simulink model "MicrogridAverage"  (R2026a)
settings: Solver=ode23t  StopTime=5  MaxStep=0.0001  RelTol=1e-4
model workspace (MAT data in the model file):
  mgIrradiance = [0  800; 1.5  800; 1.7  200; 5  200]
  mgLoadPower = [0  20000; 3.5  20000; 3.51  35000; 5  35000]
libraries: nesl_utility x20, fl_lib x9, ee_lib x8, greenH2_lib x5, batteryecm_lib x1
settings Model: Creator=LENOVO  LastModifiedBy=LENOVO
settings SimscapeCC: SimscapeLogDecimation=10.0  SimscapeLogLimitData=off

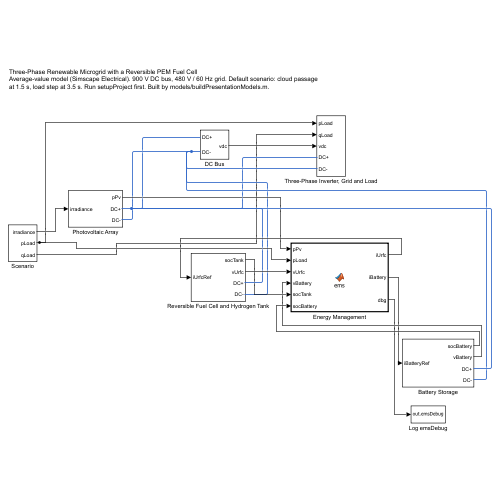
[thumbnail: Simulink's stored preview of the top-level diagram]
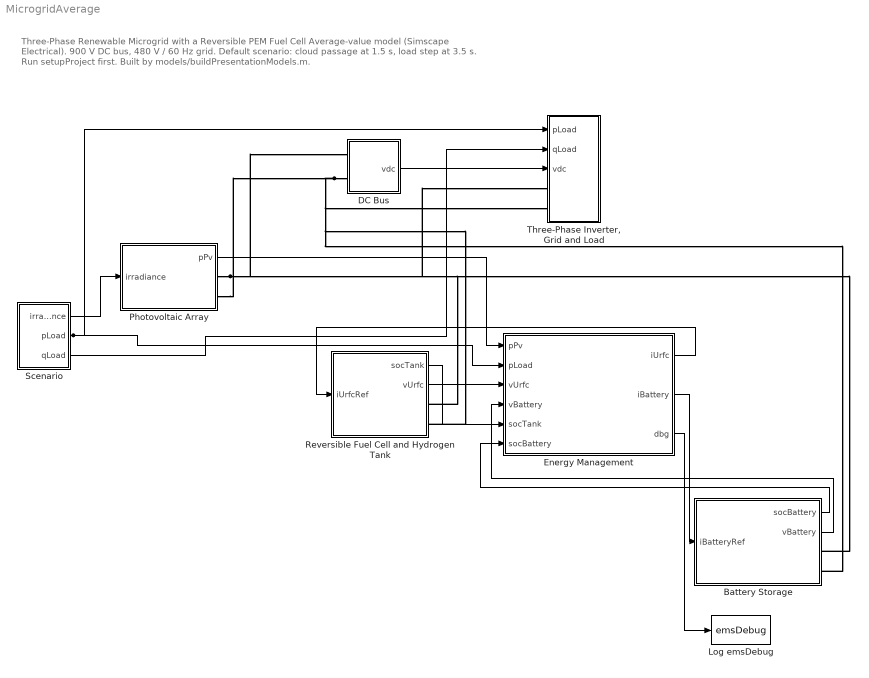
== system MicrogridAverage ==
  note: Three-Phase Renewable Microgrid with a Reversible PEM Fuel Cell
      | Average-value model (Simscape Electrical). 900 V DC bus, 480 V / 60 Hz grid. Default scenario: cloud passage
      | at 1.5 s, load step at 3.5 s. Run setupProject first. Built by models/buildPresentationModels.m.
  Battery Storage : Subsystem
  DC Bus : Subsystem
  Energy Management : MATLAB Function  TreatAsAtomicUnit=on
  Log emsDebug : ToWorkspace  VariableName=emsDebug  SaveFormat=Timeseries  SampleTime=-1
  Photovoltaic Array : Subsystem
  Reversible Fuel Cell and Hydrogen Tank : Subsystem
  Scenario : Subsystem
  "Three-Phase Inverter, Grid and Load" : Subsystem
  wires:
  Scenario/1(irradiance) -> Photovoltaic Array/1(irradiance)
  Scenario/2(pLoad) -> Energy Management/2(pLoad), "Three-Phase Inverter, Grid and Load"/1(pLoad)
  Scenario/3(qLoad) -> "Three-Phase Inverter, Grid and Load"/2(qLoad)
  DC Bus/1(vdc) -> "Three-Phase Inverter, Grid and Load"/3(vdc)
  Photovoltaic Array/1(pPv) -> Energy Management/1(pPv)
  Reversible Fuel Cell and Hydrogen Tank/1(socTank) -> Energy Management/5(socTank)
  Reversible Fuel Cell and Hydrogen Tank/2(vUrfc) -> Energy Management/3(vUrfc)
  Energy Management/1(iUrfc) -> Reversible Fuel Cell and Hydrogen Tank/1(iUrfcRef)
  Battery Storage/2(vBattery) -> Energy Management/4(vBattery)
  Energy Management/2(iBattery) -> Battery Storage/1(iBatteryRef)
  Energy Management/3(dbg) -> Log emsDebug/1
  Battery Storage/1(socBattery) -> Energy Management/6(socBattery)
  connections:
  Photovoltaic Array/RConn2 -- Reversible Fuel Cell and Hydrogen Tank/RConn2 -- "Three-Phase Inverter, Grid and Load"/LConn2 -- Battery Storage/RConn2 -- DC Bus/LConn2
  Photovoltaic Array/RConn1 -- Reversible Fuel Cell and Hydrogen Tank/RConn1 -- Battery Storage/RConn1 -- "Three-Phase Inverter, Grid and Load"/LConn1 -- DC Bus/LConn1

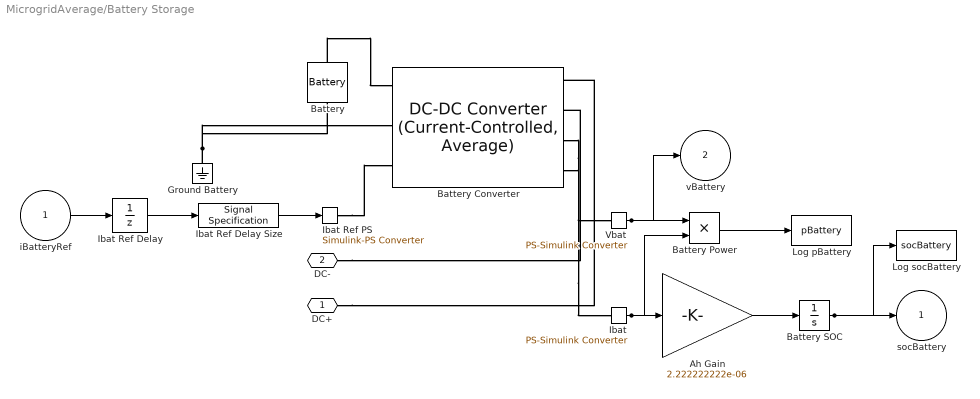
== system MicrogridAverage/Battery Storage ==
  iBatteryRef : Inport
  Ah Gain : Gain  Gain=2.222222222e-06
  Battery : batteryecm_lib/Battery  Vnom=400 V  prm_dir=simscape.enum.battery.prm_dir.disabled  R1_dis=2 Ohm  R1_ch=2 Ohm  R1=0.08 Ohm  prm_AH=simscape.enum.battery.prm_AH.finite  AH=125 A*hr  V1=380 V  AH1=62.5 A*hr  prm_R2=simscape.enum.battery.prm_R2.disabled  R2=2000 Ohm  Tmeas=298.15 K  charge_measurement_port=simscape.enum.battery.enable.no  prm_dyn=simscape.enum.battery.prm_dyn.off  Rp1=0.005 Ohm  tau1=30 s  Rp2=0.005 Ohm  tau2=30 s  Rp3=0.005 Ohm  tau3=30 s  Rp4=0.005 Ohm  tau4=30 s  Rp5=0.005 Ohm  tau5=30 s  prm_fade=simscape.enum.battery.prm_fade.disabled  N_fade=100  AH_fade=45 A*hr  R1_fade=2.02 Ohm  R1_ch_fade=2.02 Ohm  V1_fade=10.35 V  prm_age=simscape.enum.battery.prm_age.disabled  prm_age_OCV=simscape.enum.battery.prm_age_OCV.OCV  OCV_age=0.9  SOC_age=60  Tmeas_age=298.15 K  delta_time_age_vec=[0] d  temperature_age_vec=[273] K  OCV_scaling_age=2.2134e6  OCV_offset_age=1.632e6  temp_exp_age=0.515833569 V  t_exp_age=0.75  Vnom_T2=12 V  R1_T2=2.2 Ohm  R1_T2_dis=2.2 Ohm  R1_T2_ch=2.2 Ohm  V1_T2=11.4 V  R2_T2=2200 Ohm  Rp1_T2=0.005 Ohm  tau1_T2=30 s  Rp2_T2=0.005 Ohm  tau2_T2=30 s  Rp3_T2=0.005 Ohm  tau3_T2=30 s  Rp4_T2=0.005 Ohm  tau4_T2=30 s  Rp5_T2=0.005 Ohm  tau5_T2=30 s  Tmeas2=273.15 K  thermal_port=simscape.enum.thermaleffects.omit  thermal_mass=30000 J/K  i_specify=off  i_priority=None  i=0 A  i_nominal_specify=off  i_nominal_value=1  i_nominal_unit=A  v_specify=off  v_priority=None  v=0 V  v_nominal_specify=off  v_nominal_value=1  v_nominal_unit=V  charge_specify=off  charge_priority=High  charge=50 A*hr  charge_nominal_specify=off  charge_nominal_value=1  charge_nominal_unit=A*hr  num_cycles_specify=off  num_cycles_priority=High  num_cycles=0  num_cycles_nominal_specify=off  num_cycles_nominal_value=1  num_cycles_nominal_unit=1  temperature_specify=off  temperature_priority=High  temperature=298.15 K  temperature_nominal_specify=off  temperature_nominal_value=1  temperature_nominal_unit=K
  Battery Converter : greenH2_lib/DC-DC Converter (Current-Controlled, Average)  eta=0.97  v_min=10 V  i1_specify=off  i1_priority=None  i1=0 A  i1_nominal_specify=off  i1_nominal_value=1  i1_nominal_unit=A  i2_specify=off  i2_priority=None  i2=0 A  i2_nominal_specify=off  i2_nominal_value=1  i2_nominal_unit=A
  Battery Power : Product
  Battery SOC : Integrator  InitialCondition=0.6
  Ground Battery : fl_lib/Electrical/Electrical Elements/Electrical Reference
  Ibat : nesl_utility/PS-Simulink Converter  PhysicalDomain=network_engine_domain  SubClassName=ps_output  LeftPortType=input  RightPortType=output  PseudoPeriodic=off  Frequencies=[]  VectorFormat=inherit  Unit=A  AffineConversion=off
  Ibat Ref Delay : UnitDelay  SampleTime=0.001
  Ibat Ref Delay Size : SignalSpecification  Dimensions=1
  Ibat Ref PS : nesl_utility/Simulink-PS Converter  PhysicalDomain=network_engine_domain  SubClassName=ps_input  LeftPortType=input  RightPortType=output  PseudoPeriodic=off  Frequencies=[]  NoiseDistribution=none  NoiseParameters=[]  Unit=A  AffineConversion=off  FilteringAndDerivatives=provide  SimscapeFilterOrder=1  InputFilterTimeConstant=0.001  UdotUserProvided=0
  Log pBattery : ToWorkspace  VariableName=pBattery  SaveFormat=Timeseries  SampleTime=-1
  Log socBattery : ToWorkspace  VariableName=socBattery  SaveFormat=Timeseries  SampleTime=-1
  Vbat : nesl_utility/PS-Simulink Converter  PhysicalDomain=network_engine_domain  SubClassName=ps_output  LeftPortType=input  RightPortType=output  PseudoPeriodic=off  Frequencies=[]  VectorFormat=inherit  Unit=V  AffineConversion=off
  DC+ : PMIOPort  Side=Right
  DC- : PMIOPort  Port=2  Side=Right
  socBattery : Outport
  vBattery : Outport  Port=2
  wires:
  iBatteryRef/1 -> Ibat Ref Delay/1
  Ibat Ref Delay/1 -> Ibat Ref Delay Size/1
  Vbat/1 -> Battery Power/1, vBattery/1
  Ibat Ref Delay Size/1 -> Ibat Ref PS/1
  Ah Gain/1 -> Battery SOC/1
  Ibat/1 -> Ah Gain/1, Battery Power/2
  Battery Power/1 -> Log pBattery/1
  Battery SOC/1 -> socBattery/1, Log socBattery/1
  connections:
  Ground Battery/LConn1 -- Battery/RConn1 -- Battery Converter/LConn2
  Ibat Ref PS/RConn1 -- Battery Converter/LConn3
  Battery/LConn1 -- Battery Converter/LConn1
  DC-/RConn1 -- Battery Converter/RConn2
  DC+/RConn1 -- Battery Converter/RConn1
  Battery Converter/RConn4 -- Ibat/LConn1
  Battery Converter/RConn3 -- Vbat/LConn1

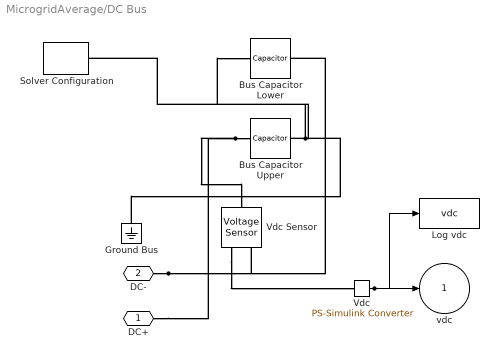
== system MicrogridAverage/DC Bus ==
  Bus Capacitor Lower : fl_lib/Electrical/Electrical Elements/Capacitor  c=0.01 F  r=1e-6 Ohm  g=0 1/Ohm  i_specify=off  i_priority=None  i=0 A  i_nominal_specify=off  i_nominal_value=1  i_nominal_unit=A  v_specify=off  v_priority=None  v=0 V  v_nominal_specify=off  v_nominal_value=1  v_nominal_unit=V  vc_specify=on  vc_priority=High  vc=450 V  vc_nominal_specify=off  vc_nominal_value=1  vc_nominal_unit=V
  Bus Capacitor Upper : fl_lib/Electrical/Electrical Elements/Capacitor  c=0.01 F  r=1e-6 Ohm  g=0 1/Ohm  i_specify=off  i_priority=None  i=0 A  i_nominal_specify=off  i_nominal_value=1  i_nominal_unit=A  v_specify=off  v_priority=None  v=0 V  v_nominal_specify=off  v_nominal_value=1  v_nominal_unit=V  vc_specify=on  vc_priority=High  vc=450 V  vc_nominal_specify=off  vc_nominal_value=1  vc_nominal_unit=V
  Ground Bus : fl_lib/Electrical/Electrical Elements/Electrical Reference
  Log vdc : ToWorkspace  VariableName=vdc  SaveFormat=Timeseries  SampleTime=-1
  Solver Configuration : nesl_utility/Solver Configuration  PhysicalDomain=network_engine_domain  SubClassName=solver  LeftPortType=input  RightPortType=generic  Tones=[]  Harmonics=[]  SimulateNoise=off  Profile=off  UseLocalSampling=off  EnableSwitchedLinearOptims=on  FrequencyDomain=off  UseCCode=off  RelTol=0.001  AbsTol=0.001  MinStep=1e-09  ToWorkspace=off  RevertToSquareIcSolve=off  NumHomotopyIterations=100  PhasorMode=off  PhasorModeNumHarmonics=1  ConsistencySolver=NEWTON_XTOL_AFTER_FTOL  CanonicalOrdering=CANONICAL  OptimizeIntermediates=OPTIMIZED  IndexReductionMethod=DerivativeReplacement  DoDC=off  ResidualTolerance=1e-09  ConsistencyTolSource=GLOBAL  ConsistencyAbsTol=0.001  ConsistencyRelTol=0.001  ConsistencyTolFactor=0.001  UseLocalSolver=off  LocalSolverChoice=NE_BACKWARD_EULER_ADVANCER  ResolveIndetEquations=on  FunctionEvalNumThread=1  LocalSolverSampleTime=0.001  DoFixedCost=off  MaxNonlinIter=3  MaxModeIter=2  ComputeImpulses=off  ImpulseIterations=2  LinearAlgebra=auto  LinearAlgebraNumThread=0  EquationFormulation=NE_TIME_EF  DelaysMemoryBudget=1024  AutomaticFiltering=on  FilteringTimeConstant=0.001  PartitionStorageMethod=AS_NEEDED  PartitionMemoryBudget=1024  PartitionMethod=ROBUST  MultibodyUseLocalSolver=off  MultibodyLocalSolverChoice=ODE1  MultibodyLocalSolverSampleTime=0.001
  Vdc : nesl_utility/PS-Simulink Converter  PhysicalDomain=network_engine_domain  SubClassName=ps_output  LeftPortType=input  RightPortType=output  PseudoPeriodic=off  Frequencies=[]  VectorFormat=inherit  Unit=V  AffineConversion=off
  Vdc Sensor : fl_lib/Electrical/Electrical Sensors/Voltage Sensor
  DC+ : PMIOPort  Side=Left
  DC- : PMIOPort  Port=2  Side=Left
  vdc : Outport
  wires:
  Vdc/1 -> Log vdc/1, vdc/1
  connections:
  Ground Bus/LConn1 -- Solver Configuration/RConn1 -- Bus Capacitor Lower/LConn1 -- Bus Capacitor Upper/RConn1
  DC-/RConn1 -- Vdc Sensor/RConn2 -- Bus Capacitor Lower/RConn1
  DC+/RConn1 -- Vdc Sensor/LConn1 -- Bus Capacitor Upper/LConn1
  Vdc Sensor/RConn1 -- Vdc/LConn1

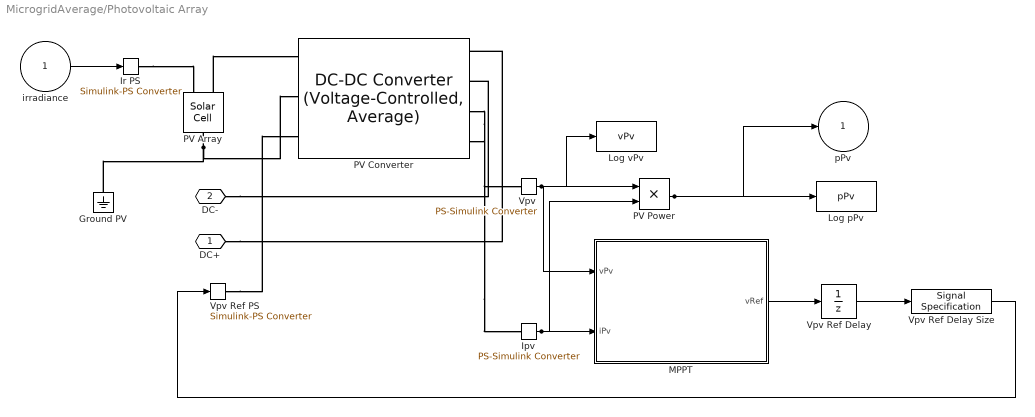
== system MicrogridAverage/Photovoltaic Array ==
  irradiance : Inport
  Ground PV : fl_lib/Electrical/Electrical Elements/Electrical Reference
  Ipv : nesl_utility/PS-Simulink Converter  PhysicalDomain=network_engine_domain  SubClassName=ps_output  LeftPortType=input  RightPortType=output  PseudoPeriodic=off  Frequencies=[]  VectorFormat=inherit  Unit=A  AffineConversion=off
  Ir PS : nesl_utility/Simulink-PS Converter  PhysicalDomain=network_engine_domain  SubClassName=ps_input  LeftPortType=input  RightPortType=output  PseudoPeriodic=off  Frequencies=[]  NoiseDistribution=none  NoiseParameters=[]  Unit=W/m^2  AffineConversion=off  FilteringAndDerivatives=provide  SimscapeFilterOrder=1  InputFilterTimeConstant=0.001  UdotUserProvided=0
  Log pPv : ToWorkspace  VariableName=pPv  SaveFormat=Timeseries  SampleTime=-1
  Log vPv : ToWorkspace  VariableName=vPv  SaveFormat=Timeseries  SampleTime=-1
  MPPT : MATLAB Function  TreatAsAtomicUnit=on
  PV Array : ee_lib/Sources/Solar Cell  prm=ee.enum.sources.solar_cell_prm.datasheet  Isc=9 A  Voc=0.6 V  Is=1e-6 A  Is2=0 A  Iph=7.34 A  Ir0=1000 W/m^2  ec=1.5  N2=2  Rs=0 Ohm  Rp=inf Ohm  N_series=1200  N_parallel=12  TIPH1=0 1/K  EG=1.11 eV  TXIS1=3  TXIS2=3  TRS1=0  TRP1=0  Tmeas=25 degC  TFIXED=25 degC  thermal_mass=100 J/K  initial_temperature=25 degC
  PV Converter : greenH2_lib/DC-DC Converter (Voltage-Controlled, Average)  eta=0.98  v_min=10 V  i1_specify=off  i1_priority=None  i1=0 A  i1_nominal_specify=off  i1_nominal_value=1  i1_nominal_unit=A  i2_specify=off  i2_priority=None  i2=0 A  i2_nominal_specify=off  i2_nominal_value=1  i2_nominal_unit=A
  PV Power : Product
  Vpv : nesl_utility/PS-Simulink Converter  PhysicalDomain=network_engine_domain  SubClassName=ps_output  LeftPortType=input  RightPortType=output  PseudoPeriodic=off  Frequencies=[]  VectorFormat=inherit  Unit=V  AffineConversion=off
  Vpv Ref Delay : UnitDelay  InitialCondition=570  SampleTime=0.01
  Vpv Ref Delay Size : SignalSpecification  Dimensions=1
  Vpv Ref PS : nesl_utility/Simulink-PS Converter  PhysicalDomain=network_engine_domain  SubClassName=ps_input  LeftPortType=input  RightPortType=output  PseudoPeriodic=off  Frequencies=[]  NoiseDistribution=none  NoiseParameters=[]  Unit=V  AffineConversion=off  FilteringAndDerivatives=provide  SimscapeFilterOrder=1  InputFilterTimeConstant=0.001  UdotUserProvided=0
  DC+ : PMIOPort  Side=Right
  DC- : PMIOPort  Port=2  Side=Right
  pPv : Outport
  wires:
  PV Power/1 -> pPv/1, Log pPv/1
  irradiance/1 -> Ir PS/1
  Vpv/1 -> MPPT/1(vPv), PV Power/1, Log vPv/1
  Ipv/1 -> MPPT/2(iPv), PV Power/2
  MPPT/1(vRef) -> Vpv Ref Delay/1
  Vpv Ref Delay/1 -> Vpv Ref Delay Size/1
  Vpv Ref Delay Size/1 -> Vpv Ref PS/1
  connections:
  Ground PV/LConn1 -- PV Array/RConn1 -- PV Converter/LConn2
  Ir PS/RConn1 -- PV Array/LConn1
  PV Array/LConn2 -- PV Converter/LConn1
  DC-/RConn1 -- PV Converter/RConn2
  DC+/RConn1 -- PV Converter/RConn1
  PV Converter/RConn4 -- Ipv/LConn1
  Vpv Ref PS/RConn1 -- PV Converter/LConn3
  PV Converter/RConn3 -- Vpv/LConn1

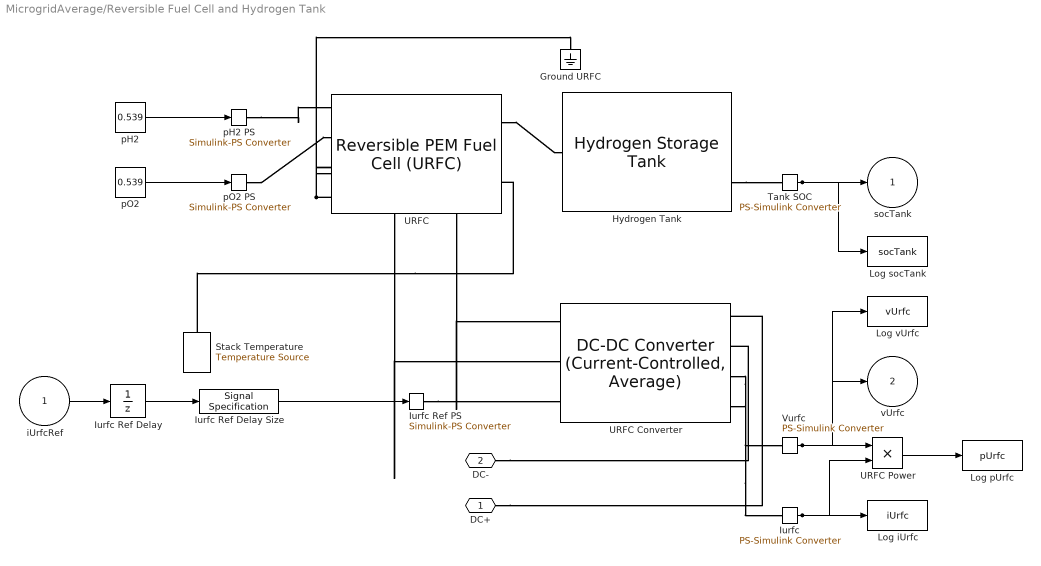
== system MicrogridAverage/Reversible Fuel Cell and Hydrogen Tank ==
  iUrfcRef : Inport
  Ground URFC : fl_lib/Electrical/Electrical Elements/Electrical Reference
  Hydrogen Tank : greenH2_lib/Hydrogen Storage Tank  V_tank=0.5 m^3  T_tank=298.15 K  p_init=30 bar  p_min=5 bar  p_max=350 bar  b_H2=1.55e-05 m^3/mol  n_specify=off  n_priority=None  n=1000 mol  n_nominal_specify=off  n_nominal_value=1  n_nominal_unit=mol
  Iurfc : nesl_utility/PS-Simulink Converter  PhysicalDomain=network_engine_domain  SubClassName=ps_output  LeftPortType=input  RightPortType=output  PseudoPeriodic=off  Frequencies=[]  VectorFormat=inherit  Unit=A  AffineConversion=off
  Iurfc Ref Delay : UnitDelay  SampleTime=0.001
  Iurfc Ref Delay Size : SignalSpecification  Dimensions=1
  Iurfc Ref PS : nesl_utility/Simulink-PS Converter  PhysicalDomain=network_engine_domain  SubClassName=ps_input  LeftPortType=input  RightPortType=output  PseudoPeriodic=off  Frequencies=[]  NoiseDistribution=none  NoiseParameters=[]  Unit=A  AffineConversion=off  FilteringAndDerivatives=provide  SimscapeFilterOrder=1  InputFilterTimeConstant=0.001  UdotUserProvided=0
  Log iUrfc : ToWorkspace  VariableName=iUrfc  SaveFormat=Timeseries  SampleTime=-1
  Log pUrfc : ToWorkspace  VariableName=pUrfc  SaveFormat=Timeseries  SampleTime=-1
  Log socTank : ToWorkspace  VariableName=socTank  SaveFormat=Timeseries  SampleTime=-1
  Log vUrfc : ToWorkspace  VariableName=vUrfc  SaveFormat=Timeseries  SampleTime=-1
  Stack Temperature : fl_lib/Thermal/Thermal Sources/Temperature Source  temperature=353.15 K
  Tank SOC : nesl_utility/PS-Simulink Converter  PhysicalDomain=network_engine_domain  SubClassName=ps_output  LeftPortType=input  RightPortType=output  PseudoPeriodic=off  Frequencies=[]  VectorFormat=inherit  Unit=1  AffineConversion=off
  URFC : greenH2_lib/Reversible PEM Fuel Cell (URFC)  N_cell=100  A_cell=300 cm^2  t_mem=0.0050800000000000003 cm  lambda_EC=22  lambda_FC=10.109999999999999  R_contact=0.037440000000000001 Ohm*cm^2  j0_EC=0.0001009 A/cm^2  alpha_EC=0.5  j0_FC=1.4800000000000001e-05 A/cm^2  alpha_FC=0.5  gamma_O2=0.75149999999999995  E_a=0 J/mol  T_ref=353.14999999999998 K  jL_EC=20 A/cm^2  jL_FC=17.780000000000001 A/cm^2  psi_H2=8.2000000000000001e-11 mol/(cm*s*bar)  i_specify=off  i_priority=None  i=0 A  i_nominal_specify=off  i_nominal_value=1  i_nominal_unit=A  Q_specify=off  Q_priority=None  Q=0 W  Q_nominal_specify=off  Q_nominal_value=1  Q_nominal_unit=W
  URFC Converter : greenH2_lib/DC-DC Converter (Current-Controlled, Average)  eta=0.97  v_min=10 V  i1_specify=off  i1_priority=None  i1=0 A  i1_nominal_specify=off  i1_nominal_value=1  i1_nominal_unit=A  i2_specify=off  i2_priority=None  i2=0 A  i2_nominal_specify=off  i2_nominal_value=1  i2_nominal_unit=A
  URFC Power : Product
  Vurfc : nesl_utility/PS-Simulink Converter  PhysicalDomain=network_engine_domain  SubClassName=ps_output  LeftPortType=input  RightPortType=output  PseudoPeriodic=off  Frequencies=[]  VectorFormat=inherit  Unit=V  AffineConversion=off
  pH2 : Constant  Value=0.539
  pH2 PS : nesl_utility/Simulink-PS Converter  PhysicalDomain=network_engine_domain  SubClassName=ps_input  LeftPortType=input  RightPortType=output  PseudoPeriodic=off  Frequencies=[]  NoiseDistribution=none  NoiseParameters=[]  Unit=bar  AffineConversion=off  FilteringAndDerivatives=provide  SimscapeFilterOrder=1  InputFilterTimeConstant=0.001  UdotUserProvided=0
  pO2 : Constant  Value=0.539
  pO2 PS : nesl_utility/Simulink-PS Converter  PhysicalDomain=network_engine_domain  SubClassName=ps_input  LeftPortType=input  RightPortType=output  PseudoPeriodic=off  Frequencies=[]  NoiseDistribution=none  NoiseParameters=[]  Unit=bar  AffineConversion=off  FilteringAndDerivatives=provide  SimscapeFilterOrder=1  InputFilterTimeConstant=0.001  UdotUserProvided=0
  DC+ : PMIOPort  Side=Right
  DC- : PMIOPort  Port=2  Side=Right
  socTank : Outport
  vUrfc : Outport  Port=2
  wires:
  Iurfc Ref Delay/1 -> Iurfc Ref Delay Size/1
  iUrfcRef/1 -> Iurfc Ref Delay/1
  pH2/1 -> pH2 PS/1
  pO2/1 -> pO2 PS/1
  Iurfc Ref Delay Size/1 -> Iurfc Ref PS/1
  Iurfc/1 -> Log iUrfc/1, URFC Power/2
  Tank SOC/1 -> socTank/1, Log socTank/1
  Vurfc/1 -> vUrfc/1, URFC Power/1, Log vUrfc/1
  URFC Power/1 -> Log pUrfc/1
  connections:
  URFC Converter/RConn3 -- Vurfc/LConn1
  URFC/LConn4 -- URFC Converter/LConn2 -- Ground URFC/LConn1
  pH2 PS/RConn1 -- URFC/LConn1
  DC-/RConn1 -- URFC Converter/RConn2
  pO2 PS/RConn1 -- URFC/LConn2
  URFC Converter/RConn4 -- Iurfc/LConn1
  Stack Temperature/LConn1 -- URFC/RConn2
  URFC/RConn1 -- Hydrogen Tank/LConn1
  URFC/LConn3 -- URFC Converter/LConn1
  Iurfc Ref PS/RConn1 -- URFC Converter/LConn3
  DC+/RConn1 -- URFC Converter/RConn1
  Hydrogen Tank/RConn2 -- Tank SOC/LConn1

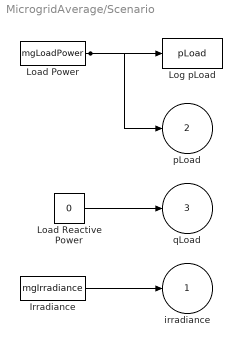
== system MicrogridAverage/Scenario ==
  Irradiance : FromWorkspace  VariableName=mgIrradiance  OutputAfterFinalValue=Holding final value
  Load Power : FromWorkspace  VariableName=mgLoadPower  OutputAfterFinalValue=Holding final value
  Load Reactive Power : Constant  Value=0
  Log pLoad : ToWorkspace  VariableName=pLoad  SaveFormat=Timeseries  SampleTime=-1
  irradiance : Outport
  pLoad : Outport  Port=2
  qLoad : Outport  Port=3
  wires:
  Irradiance/1 -> irradiance/1
  Load Power/1 -> pLoad/1, Log pLoad/1
  Load Reactive Power/1 -> qLoad/1

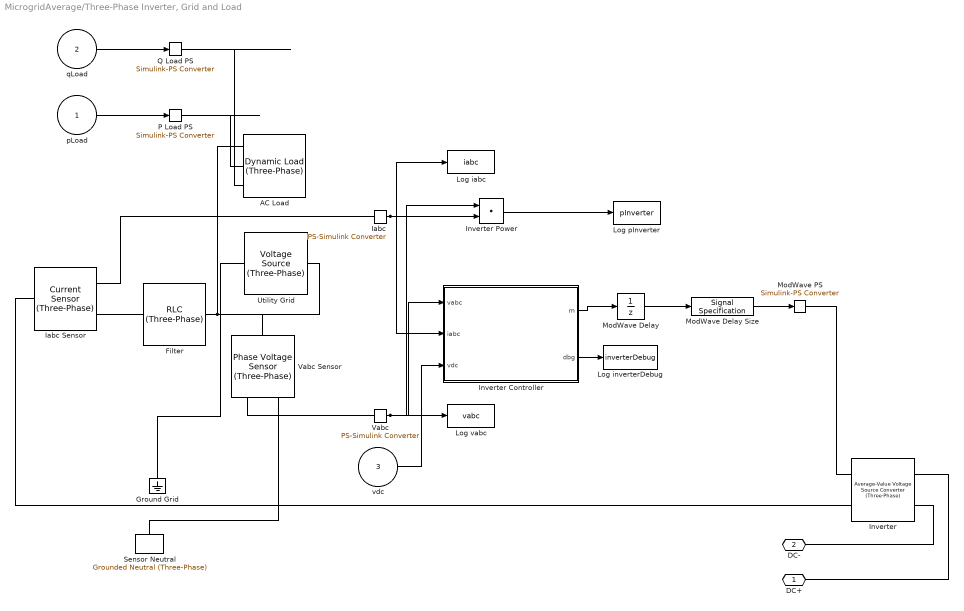
== system MicrogridAverage/Three-Phase Inverter, Grid and Load ==
  pLoad : Inport
  qLoad : Inport  Port=2
  vdc : Inport  Port=3
  AC Load : ee_lib/Passive/Dynamic Load (Three-Phase)  port_option=ee.enum.threePhasePort.composite  FRated=60 Hz  Vline_rms_min=240 V  tau=0.01 s  Vline_rms_ini=480 V  Vang_ini=0 deg  gmin=0 S
  Filter : ee_lib/Passive/RLC Assemblies/RLC (Three-Phase)  port_option=ee.enum.threePhasePort.composite  component_structure=ee.enum.rlc.structure.SeriesRL  R=0.05 Ohm  L=0.002 H  C=1e-6 F  R_parasitic=0 Ohm  G_parasitic=0 1/Ohm  IL_specify=off  IL_priority=High  IL=[0, 0, 0] A  IL_nominal_specify=off  IL_nominal_value=1  IL_nominal_unit=A  VC_specify=off  VC_priority=High  VC=[0, 0, 0] V  VC_nominal_specify=off  VC_nominal_value=1  VC_nominal_unit=V
  Ground Grid : fl_lib/Electrical/Electrical Elements/Electrical Reference
  Iabc : nesl_utility/PS-Simulink Converter  PhysicalDomain=network_engine_domain  SubClassName=ps_output  LeftPortType=input  RightPortType=output  PseudoPeriodic=off  Frequencies=[]  VectorFormat=inherit  Unit=A  AffineConversion=off
  Iabc Sensor : ee_lib/Sensors & Transducers/Current Sensor (Three-Phase)  port_option=ee.enum.threePhasePort.composite
  Inverter : ee_lib/Semiconductors & Converters/Converters/Average-Value Voltage Source Converter (Three-Phase)  port_option=ee.enum.threePhasePort.composite  enable_block_pulses_input=false  krec=0.01 Ohm  frequency_option=ee.enum.converters.frequency.variable  input_option=ee.enum.converters.inputOption.ModWave  FRated=60 Hz  losses_parameterization=ee.enum.converters.losses.fixed  Pfixed=1 W  ks=0.01  kc1=1.7 V  kc2=0.01 Ohm  Ploss_vect=[100, 800, 1870, 3250, 4900] W  Irms_vect=[10, 100, 200, 300, 400] A  Vdc_nom=300 V  thermal_mass=30000 J/K  temperature_specify=off  temperature_priority=High  temperature=298.15 K  temperature_nominal_specify=off  temperature_nominal_value=1  temperature_nominal_unit=K
  Inverter Controller : MATLAB Function  TreatAsAtomicUnit=on
  Inverter Power : DotProduct  OutDataTypeStr=Inherit: Inherit via internal rule
  Log iabc : ToWorkspace  VariableName=iabc  SaveFormat=Timeseries  SampleTime=-1
  Log inverterDebug : ToWorkspace  VariableName=inverterDebug  SaveFormat=Timeseries  SampleTime=-1
  Log pInverter : ToWorkspace  VariableName=pInverter  SaveFormat=Timeseries  SampleTime=-1
  Log vabc : ToWorkspace  VariableName=vabc  SaveFormat=Timeseries  SampleTime=-1
  ModWave Delay : UnitDelay  InitialCondition=[0;0;0]  SampleTime=0.0001
  ModWave Delay Size : SignalSpecification  Dimensions=[3 1]
  ModWave PS : nesl_utility/Simulink-PS Converter  PhysicalDomain=network_engine_domain  SubClassName=ps_input  LeftPortType=input  RightPortType=output  PseudoPeriodic=off  Frequencies=[]  NoiseDistribution=none  NoiseParameters=[]  Unit=1  AffineConversion=off  FilteringAndDerivatives=provide  SimscapeFilterOrder=1  InputFilterTimeConstant=0.001  UdotUserProvided=0
  P Load PS : nesl_utility/Simulink-PS Converter  PhysicalDomain=network_engine_domain  SubClassName=ps_input  LeftPortType=input  RightPortType=output  PseudoPeriodic=off  Frequencies=[]  NoiseDistribution=none  NoiseParameters=[]  Unit=W  AffineConversion=off  FilteringAndDerivatives=provide  SimscapeFilterOrder=1  InputFilterTimeConstant=0.001  UdotUserProvided=0
  Q Load PS : nesl_utility/Simulink-PS Converter  PhysicalDomain=network_engine_domain  SubClassName=ps_input  LeftPortType=input  RightPortType=output  PseudoPeriodic=off  Frequencies=[]  NoiseDistribution=none  NoiseParameters=[]  Unit=V*A  AffineConversion=off  FilteringAndDerivatives=provide  SimscapeFilterOrder=1  InputFilterTimeConstant=0.001  UdotUserProvided=0
  Sensor Neutral : ee_lib/Connectors & References/Grounded Neutral (Three-Phase)  port_option=ee.enum.threePhasePort.composite
  Utility Grid : ee_lib/Sources/Voltage Source (Three-Phase)  vline_rms=480 V  shift=0 deg  freq=60 Hz  impedance_option=0  SShortCircuit=1e6 A*V  XR=15  R=0.01 Ohm  L=3.97e-4 H  harmonic_option=0  harmonic_orders=[5, 7, 11, 13]  harmonic_ratios=[.1, .1, .1, .1]  G_parasitic=0 1/Ohm  I_specify=off  I_priority=None  I=[0, 0, 0] A  I_nominal_specify=off  I_nominal_value=1  I_nominal_unit=A
  Vabc : nesl_utility/PS-Simulink Converter  PhysicalDomain=network_engine_domain  SubClassName=ps_output  LeftPortType=input  RightPortType=output  PseudoPeriodic=off  Frequencies=[]  VectorFormat=inherit  Unit=V  AffineConversion=off
  Vabc Sensor : ee_lib/Sensors & Transducers/Phase Voltage Sensor (Three-Phase)  port_option=ee.enum.threePhasePort.composite
  DC+ : PMIOPort  Side=Left
  DC- : PMIOPort  Port=2  Side=Left
  wires:
  qLoad/1 -> Q Load PS/1
  pLoad/1 -> P Load PS/1
  Iabc/1 -> Inverter Controller/2(iabc), Log iabc/1, Inverter Power/2
  Vabc/1 -> Inverter Power/1, Inverter Controller/1(vabc), Log vabc/1
  vdc/1 -> Inverter Controller/3(vdc)
  Inverter Power/1 -> Log pInverter/1
  Inverter Controller/1(m) -> ModWave Delay/1
  Inverter Controller/2(dbg) -> Log inverterDebug/1
  ModWave Delay/1 -> ModWave Delay Size/1
  ModWave Delay Size/1 -> ModWave PS/1
  connections:
  ModWave PS/RConn1 -- Inverter/LConn1
  Iabc Sensor/LConn1 -- Inverter/LConn2
  Q Load PS/RConn1 -- AC Load/LConn3
  Vabc Sensor/RConn1 -- Vabc/LConn1
  Iabc Sensor/RConn2 -- Filter/LConn1
  Filter/RConn1 -- Vabc Sensor/LConn1 -- Utility Grid/RConn1 -- AC Load/LConn1
  Iabc Sensor/RConn1 -- Iabc/LConn1
  P Load PS/RConn1 -- AC Load/LConn2
  Ground Grid/LConn1 -- Utility Grid/LConn1
  Sensor Neutral/LConn1 -- Vabc Sensor/RConn2
  DC-/RConn1 -- Inverter/RConn2
  DC+/RConn1 -- Inverter/RConn1

== matlab function MicrogridAverage/Three-Phase Inverter, Grid and Load/Inverter Controller ==
  settings: updateMethod=DISCRETE  sampleTime=0.0001
  data: vabc input double size=3; m output double size=[3 1]; iabc input double size=3; vdc input double size=1; dbg output double size=[6 1]
function [m, dbg] = inverterController(vabc, iabc, vdc)
%#codegen
% Grid-following control regulating the DC bus (microgrid.inverterControlStep)
persistent state
p = microgrid.controlParameters();
if isempty(state)
    state = zeros(5, 1);
end
[m, state, dbg] = microgrid.inverterControlStep(vabc(:), iabc(:), vdc, state, p);
end

== matlab function MicrogridAverage/Energy Management ==
  settings: updateMethod=DISCRETE  sampleTime=0.001
  data: pPv input double size=1; iUrfc output double size=1; pLoad input double size=1; vUrfc input double size=1; vBattery input double size=1; socTank input double size=1; socBattery input double size=1; iBattery output double size=1; dbg output double size=[4 1]
function [iUrfc, iBattery, dbg] = ems(pPv, pLoad, vUrfc, vBattery, socTank, socBattery)
%#codegen
% Rule-based power sharing between URFC and battery (microgrid.emsStep)
persistent state
p = microgrid.controlParameters();
if isempty(state)
    state = 0;
end
[iUrfc, iBattery, state, dbg] = microgrid.emsStep(pPv, pLoad, vUrfc, vBattery, socTank, socBattery, state, p);
end

== matlab function MicrogridAverage/Photovoltaic Array/MPPT ==
  settings: updateMethod=DISCRETE  sampleTime=0.01
  data: vPv input double size=1; vRef output double size=1; iPv input double size=1
function vRef = mppt(vPv, iPv)
%#codegen
% Perturb-and-observe maximum power point tracking (microgrid.mpptStep)
persistent state
p = microgrid.controlParameters();
if isempty(state)
    state = [p.vMpptInit; 0; 1];
end
[vRef, state] = microgrid.mpptStep(vPv, iPv, state, p);
end
